simulink model "model"  (R2024b)
settings: Solver=FixedStepDiscrete  StartTime=0.0  StopTime=30  FixedStep=0.1  RelTol=1e-3  EnableMultiTasking=on
libraries: stm32f4xxblockslib x6, stm32g4xxblockslib x2, stm32blockslib x2
(part 1 of 2)
settings Model: STM32="{\"DigitalPortWrite\":[{\"ID\":\"project:49\"},{\"ID\":\"project:50\"},{\"ID\":\"model:49\"},{\"ID\":\"model:50\"}],\"DigitalPortRead\":[{\"ID\":\"project:51\"},{\"ID\":\"project:56\"},{\"ID\":\"project:78\"},{\"ID\":\"project:79\"},{\"ID\":\"model:51\"},{\"ID\":\"model:56\"},{\"ID\":\"model:78\"},{\"ID\":\"model:79\"}],\"UARTWrite\":[{\"ID\":\"project:53\"},{\"ID\":\"model:53\"}],\"UARTRead\":[{\"ID\":\"project:64\"},{\"ID\":\"model:64\"}],\"PWMOutput\":[{\"ID\":\"project:84\"},{\"ID\":\"project:87\"},{\"ID\":\"model:84\"},{\"ID\":\"model:87\"}]}"  PacingRate=5  Creator=Altair  LastModifiedBy=Altair
settings SolverCC: AlgebraicLoopSolver=TrustRegion  AutoInsertRateTranBlk=on
settings DataIOCC: LimitDataPoints=on
settings OptimizationCC: DefaultParameterBehavior=Inlined  EnhancedBackFolding=on  PassReuseOutputArgsAs=Individual arguments  ZeroExternalMemoryAtStartup=off  ZeroInternalMemoryAtStartup=off  MaxStackSize=512  OptimizeBlockOrder=speed  DifferentSizesBufferReuse=on  OptimizationCustomize=off  EfficientTunableParamExpr=on
settings DebuggingCC: ParameterTunabilityLossMsg=error  UnconnectedInputMsg=warning  UnconnectedOutputMsg=warning  UnconnectedLineMsg=warning  AllowSymbolicDim=off  SFUnexpectedBacktrackingDiag=warning  SFNoUnconditionalDefaultTransitionDiag=warning  SFExecutionAtInitializationDiag=none  ArithmeticOperatorsInVariantConditions=warning
settings HardwareCC: ProdBitPerPointer=32  ProdBitPerSizeT=32  ProdBitPerPtrDiffT=32  ProdLargestAtomicInteger=Long  ProdLargestAtomicFloat=Double  ProdWordSize=32  ProdLongLongMode=on  ProdHWDeviceType=ARM Compatible->ARM Cortex-M
settings ModelReferenceCC: EnableRefExpFcnMdlSchedulingChecks=on
settings SFSimCC: SimUseLocalCustomCode=off  CustomCodeUndefinedFunction=UseInterfaceOnly
settings RTWCC: Description=Embedded Coder  SystemTargetFile=ert.tlc  HardwareBoard=STM32G4xx Based  TemplateMakefile=ert_default_tmf  RTWUseLocalCustomCode=off  Toolchain=GNU Tools for ARM Embedded Processors  GPUComputeCapability=3.5  DLArmComputeVersion=19.05
settings CodeAppCC: ForceParamTrailComments=on  IgnoreCustomStorageClasses=off  OperatorAnnotations=on  SimulinkDataObjDesc=on  SFDataObjDesc=on  InsertBlockDesc=on
settings ERTTargetCC: TargetLangStandard=C99 (ISO)  CodeReplacementLibrary=ARM Cortex-M  ExtModeTransport=3  ExtModeStaticAlloc=on  ExtModeStaticAllocSize=2048  ExtModeMexFile=ext_xcp  ExtModeIntrfLevel=Level2 - Open
settings ConfigComp: CovMetricSettings=dw  CovSaveCumulativeToWorkspaceVar=on  CovSaveSingleToWorkspaceVar=on  CovExternalEMLEnable=off  CovSFcnEnable=off

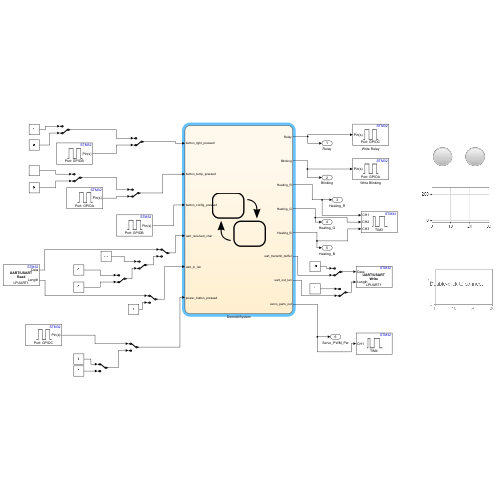
[thumbnail: Simulink's stored preview of the top-level diagram]
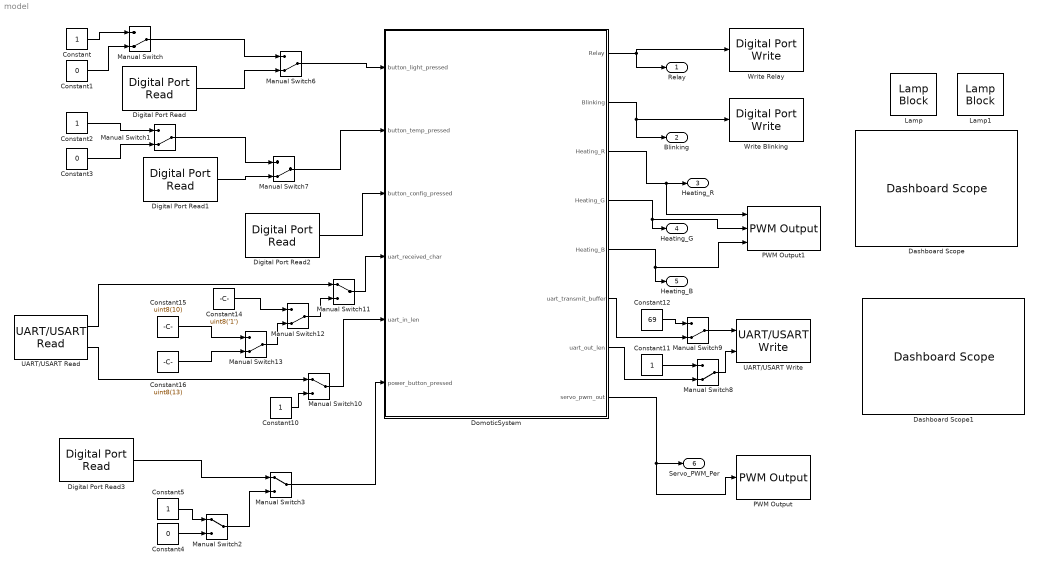
== system model ==
  Constant : Constant  OutDataTypeStr=boolean
  Constant1 : Constant  Value=0  OutDataTypeStr=boolean
  Constant10 : Constant  OutDataTypeStr=uint8
  Constant11 : Constant  OutDataTypeStr=uint8
  Constant12 : Constant  Value=69  OutDataTypeStr=uint8
  Constant14 : Constant  Value=uint8('1')  OutDataTypeStr=uint8
  Constant15 : Constant  Value=uint8(10)  OutDataTypeStr=uint8
  Constant16 : Constant  Value=uint8(13)  OutDataTypeStr=uint8
  Constant2 : Constant  OutDataTypeStr=boolean
  Constant3 : Constant  Value=0  OutDataTypeStr=boolean
  Constant4 : Constant  Value=0  OutDataTypeStr=boolean
  Constant5 : Constant  OutDataTypeStr=boolean
  Dashboard Scope : DashboardScope  Ymin=-10  Ymax=256
  Dashboard Scope1 : DashboardScope  Ymin=0  Ymax=15
  Digital Port Read : stm32f4xxblockslib/Digital Port Read  PortName=GPIOB  PinNumber=[1]  ReadOperation=on  IOAsArray=on  SampleTime=-1  EnableSimPort=off  hoistedMaskSrc=ECSoC/ECSimCodegen/Digital Port Read
      settings: LibrarySourceBlock=stm32g4xxblockslib/Digital Port Read
  Digital Port Read1 : stm32f4xxblockslib/Digital Port Read  PortName=GPIOA  PinNumber=[15]  ReadOperation=on  IOAsArray=on  SampleTime=-1  EnableSimPort=off  hoistedMaskSrc=ECSoC/ECSimCodegen/Digital Port Read
      settings: LibrarySourceBlock=stm32g4xxblockslib/Digital Port Read
  Digital Port Read2 : stm32f4xxblockslib/Digital Port Read  PortName=GPIOB  PinNumber=[0]  ReadOperation=on  IOAsArray=on  SampleTime=-1  EnableSimPort=off  hoistedMaskSrc=ECSoC/ECSimCodegen/Digital Port Read
      settings: LibrarySourceBlock=stm32g4xxblockslib/Digital Port Read
  Digital Port Read3 : stm32f4xxblockslib/Digital Port Read  PortName=GPIOC  PinNumber=[13]  ReadOperation=on  IOAsArray=on  SampleTime=-1  EnableSimPort=off  hoistedMaskSrc=ECSoC/ECSimCodegen/Digital Port Read
      settings: LibrarySourceBlock=stm32g4xxblockslib/Digital Port Read
  DomoticSystem : Stateflow chart  TreatAsAtomicUnit=on
      settings: PortSchema="{\"entries\":[{\"content\":{\"sides\":[{\"content\":{\"connectorIds\":[\"In1\",\"In2\",\"In3\",\"In4\",\"In5\",\"In6\"]},\"type\":\"ConnectorPlacement.EquallySpacedRectSide\",\"uuid\":\"9804a8b5-515a-4f98-bc64-60622ecf1453\"},{\"content\":{\"connectorIds\":[\"Out1\",\"Out2\",\"Out4\",\"Out5\",\"Out3\",\"Out6\",\"Out7\",\"Out8\"],\"side\":\"RIGHT\"},\"type\":\"ConnectorPlacement.EquallySpacedRectSide\",\"uuid\":\"716347a5-6ea0-4d99-9cb4-efcd0cc8ed47\"},{\"content\":{\"side\":\"TOP\"},\"type\":\"ConnectorPlacement.EquallySpacedRectSide\",\"uuid\":\"ac427371-1bdc-47f0-96c4-0f31dbc467ea\"}]},\"type\":\"ConnectorPlacement.EquallySpacedConnector\",\"uuid\":\"093d2936-03b8-406c-962a-bf339fa06041\"}],\"packageUris\":[\"http://schema.mathworks.com/mf0/Connector/R2020b\"],\"version\":\"1.0\"}"
  Lamp : LampBlock  LabelPosition=Hide
  Lamp1 : LampBlock  LabelPosition=Hide
  Manual Switch{,1,6..9,12..13} (8 alike) : ManualSwitch  CurrentSetting=0
  Manual Switch{2..3,10..11} (4 alike) : ManualSwitch
  PWM Output : stm32g4xxblockslib/PWM Output  TimerModule=TIM4  DutycycleUnits=Counts  EnableChannel1=on  EnableChannel2=off  EnableChannel3=off  EnableChannel4=off  EnableChannel5=off  EnableChannel6=off  EnableCounterInput=off  EnableMainOutputInput=off  EnableFrequencyInput=off  SetRCAfterCE=off  OutputDirection=off  OutputMainOutputEnableStatus=off  SampleTime=0.1  EnableSimPort=off  EnableUpdateEvent=off  EnableCaptureCompare1Event=off  EnableCaptureCompare2Event=off  EnableCaptureCompare3Event=off  EnableCaptureCompare4Event=off  EnableTriggerEvent=off  EnableBreakEvent=off  EnableBreakEvent2=off  ProcessorFamily=STM32G4  hoistedMaskSrc=ECSoC/ECSimCodegen/PWM Output
  PWM Output1 : stm32g4xxblockslib/PWM Output  TimerModule=TIM3  DutycycleUnits=Counts  EnableChannel1=on  EnableChannel2=on  EnableChannel3=on  EnableChannel4=off  EnableChannel5=off  EnableChannel6=off  EnableCounterInput=off  EnableMainOutputInput=off  EnableFrequencyInput=off  SetRCAfterCE=off  OutputDirection=off  OutputMainOutputEnableStatus=off  SampleTime=0.1  EnableSimPort=off  EnableUpdateEvent=off  EnableCaptureCompare1Event=off  EnableCaptureCompare2Event=off  EnableCaptureCompare3Event=off  EnableCaptureCompare4Event=off  EnableTriggerEvent=off  EnableBreakEvent=off  EnableBreakEvent2=off  ProcessorFamily=STM32G4  hoistedMaskSrc=ECSoC/ECSimCodegen/PWM Output
  UART/USART Read : stm32blockslib/UART//USART Read  UARTModule=LPUART1  DataType=uint8  DataLength=1  BlockingMode=off  BlockingTimeout=0.1  OutputLength=on  OutputStatus=off  SampleTime=-1
      settings: LibrarySourceBlock=stm32g4xxblockslib/UART//USART Read
  UART/USART Write : stm32blockslib/UART//USART Write  UARTModule=LPUART1  LengthOfDataToSend=on  BlockingMode=off  BlockingTimeout=0.5  OutputStatus=off
      settings: LibrarySourceBlock=stm32g4xxblockslib/UART//USART Write
  Write Blinking : stm32f4xxblockslib/Digital Port Write  PortName=GPIOA  PinNumber=[5]  ReadOperation=off  IOAsArray=on  EnableSimPort=off  hoistedMaskSrc=ECSoC/ECSimCodegen/Digital Port Write
      settings: LibrarySourceBlock=stm32g4xxblockslib/Digital Port Write
  Write Relay : stm32f4xxblockslib/Digital Port Write  PortName=GPIOC  PinNumber=[2]  ReadOperation=off  IOAsArray=on  EnableSimPort=off  hoistedMaskSrc=ECSoC/ECSimCodegen/Digital Port Write
      settings: LibrarySourceBlock=stm32g4xxblockslib/Digital Port Write
  Relay : Outport
  Blinking : Outport  Port=2
  Heating_R : Outport  Port=3
  Heating_G : Outport  Port=4
  Heating_B : Outport  Port=5
  Servo_PWM_Per : Outport  Port=6
  wires:
  Constant/1 -> Manual Switch/1
  Constant1/1 -> Manual Switch/2
  DomoticSystem/1(Relay) -> Write Relay/1, Relay/1
  Manual Switch/1 -> Manual Switch6/1
  Constant3/1 -> Manual Switch1/2
  Constant2/1 -> Manual Switch1/1
  Manual Switch1/1 -> Manual Switch7/1
  DomoticSystem/2(Blinking) -> Blinking/1, Write Blinking/1
  DomoticSystem/4(Heating_R) -> PWM Output1/1, Heating_R/1
  DomoticSystem/5(Heating_G) -> PWM Output1/2, Heating_G/1
  DomoticSystem/3(Heating_B) -> PWM Output1/3, Heating_B/1
  DomoticSystem/8(servo_pwm_out) -> PWM Output/1, Servo_PWM_Per/1
  Digital Port Read/1 -> Manual Switch6/2
  Manual Switch6/1 -> DomoticSystem/1(button_light_pressed)
  Digital Port Read1/1 -> Manual Switch7/2
  Manual Switch7/1 -> DomoticSystem/2(button_temp_pressed)
  Manual Switch8/1 -> UART/USART Write/2
  Constant11/1 -> Manual Switch8/1
  Constant12/1 -> Manual Switch9/1
  Manual Switch9/1 -> UART/USART Write/1
  UART/USART Read/1 -> Manual Switch11/1
  DomoticSystem/6(uart_transmit_buffer) -> Manual Switch9/2
  Digital Port Read2/1 -> DomoticSystem/3(button_config_pressed)
  DomoticSystem/7(uart_out_len) -> Manual Switch8/2
  UART/USART Read/2 -> Manual Switch10/1
  Manual Switch10/1 -> DomoticSystem/5(uart_in_len)
  Constant10/1 -> Manual Switch10/2
  Manual Switch11/1 -> DomoticSystem/4(uart_received_char)
  Constant14/1 -> Manual Switch12/1
  Manual Switch12/1 -> Manual Switch11/2
  Manual Switch13/1 -> Manual Switch12/2
  Constant15/1 -> Manual Switch13/1
  Constant16/1 -> Manual Switch13/2
  Digital Port Read3/1 -> Manual Switch3/1
  Constant4/1 -> Manual Switch2/2
  Manual Switch2/1 -> Manual Switch3/2
  Manual Switch3/1 -> DomoticSystem/6(power_button_pressed)
  Constant5/1 -> Manual Switch2/1
